simulink library "casper_library_reorder"  (Simulink 7.2)
settings: Solver=ode45  SolverMode=SingleTasking  StartTime=0.0  StopTime=10.0  RelTol=1e-3
libraries: xbsIndex_r4 x122, casper_library_delays x4, xps_library x2, casper_library_bus x2, casper_library_misc x1
(part 1 of 2)
settings Model: Creator=mdexter  LastModifiedBy=davidm

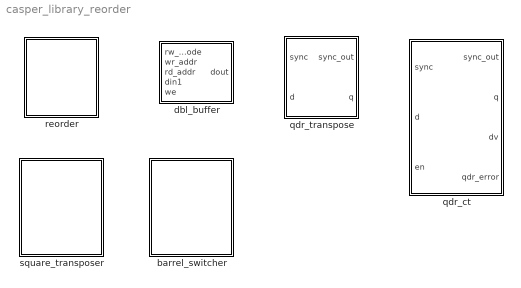
== system casper_library_reorder ==
  barrel_switcher : Subsystem  mask(barrel_switcher){n_inputs=0, async=off}
      mask prompts: n_inputs "Number of Inputs: (2^?)"; async "Asynchronous operation"
      mask help:
      | Shifts input to right by amount specified on sel,
      | wrapping around into higher order bits.
      mask init:
      | barrel_switcher_init(gcb,...
      |     'n_inputs', n_inputs, ...
      |     'async', async);
      mask Help: eval('xlWeb(''http://casper.berkeley.edu/wiki/Barrel_switcher'')')
  dbl_buffer : Subsystem  mask(dbl_buffer){depth=32, latency=2}
  qdr_ct : Subsystem  mask{idepth=10, odepth=7, which_qdr=qdr0, swap_input=no, output_order=in order, step_bits=0, custom_map=[1  15   5   7  10  14   6   0   8   9   2  13  12  11   4   3]}
      mask prompts: idepth "Input vector length (2^?)"; odepth "Output vector length (2^?)"; which_qdr "QDR SRAM chip"; swap_input "Swap input halves?"; output_order "Output column order"; step_bits "Interleave step (2^?)"; custom_map "Custom map"
      mask help:
      | Writes vectors in as rows in matrix and reads
      | out columns. Order in which columns read out
      | determined by 'Output column order' parameter.
      mask init:
      | if (strcmp(output_order, 'interleaved') == 1) && (step_bits > (idepth-1)) ,
      |     errmsg = sprintf('Can''t make step size (%i) bigger than (input vector bit size (%i) - 1)', step_bits, idepth);
      |     errordlg(errmsg);
      | end    
      | 
      | if strcmp(output_order, 'custom') && (...
      |         length(unique(custom_map)) ~= 2^idepth ||...
      |         ~isempty(find(custom_map < 0)) || ...
      |         ~isempty(find(custom_map > (2^idepth)-1))),
      |     disp('Custom map elements must be unique in range 0->2^(input vector)-1');
      |     return;
      | end
      | 
      | % set up output order (in order, interleaved, or custom)
      | map = 0 : (2^idepth)-1;
      | if strcmp(swap_input, 'yes'),
      |     map = [map((length(map)/2)+1:end), map(1:length(map)/2)];
      | end
      | if strcmp(output_order, 'interleaved'),
      |     index = zeros(1, 2^idepth);
      |     step_size = 2^(idepth-step_bits);
      |     for ctr = 0:(2^step_bits)-1,
      |         start = (ctr * step_size) + 1;
      |         finish = start + step_size - 1;
      |         index(start:finish) = ctr+1 : 2^step_bits : 2^idepth;
      |     end
      |     map = map(index);
      |     clear index;
      | elseif strcmp(output_order, 'custom'),
      |     map = map(custom_map+1);
      | end
      | 
      | %generate map so that two samples from same position in 
      | %subsequent input vectors are written into same address
      | map = reshape([map; 2^idepth+map], 1, 2^(idepth+1));
      | 
      | set_param([gcb, '/reorder'], ...
      |     'map', ['[',num2str(map),']']);
      | set_param([gcb, '/qdr'], 'which_qdr', which_qdr);
      mask StyleString: edit,edit,popup(qdr0|qdr1|qdr2|qdr3),popup(no|yes),popup(in order|interleaved|custom),edit,edit
  qdr_transpose : Subsystem  mask{idepth=9, odepth=9, which_qdr=qdr1}
      mask prompts: idepth "Input blocksize (2^n)"; odepth "Output blocksize (2^n)"; which_qdr "QDR Chip"
      mask init:
      | set_param([gcb, '/qdr'], 'which_qdr', which_qdr);
      mask StyleString: edit,edit,popup(qdr0|qdr1|qdr2|qdr3)
  reorder : Subsystem  mask(reorder){map=[], n_bits=0, n_inputs=1, bram_latency=1, map_latency=1, fanout_latency=0, double_buffer=0, bram_map=off}
      mask prompts: map "Output Order:"; n_bits "Data width in"; n_inputs "Number of inputs"; bram_latency "BRAM Latency"; map_latency "Map Latency"; fanout_latency "Fanout latency"; double_buffer "Double Buffer"; bram_map "Use BlockRAM for Map"
      mask init:
      | reorder_init(gcb, ...
      |     'map', map, ...
      |     'n_bits', n_bits, ...
      |     'n_inputs', n_inputs, ...
      |     'bram_latency', bram_latency, ...
      |     'map_latency', map_latency, ...
      |     'fanout_latency', fanout_latency, ...
      |     'double_buffer', double_buffer, ...
      |     'bram_map', bram_map);
      mask Help: eval('xlWeb(''http://casper.berkeley.edu/wiki/Reorder'')')
  square_transposer : Subsystem  mask(square_transposer){n_inputs=0, async=off}
      mask prompts: n_inputs "Number of inputs (2^?):"; async "Aynchronus operation"
      mask init:
      | square_transposer_init(gcb,...
      |     'n_inputs', n_inputs, ...
      |     'async', async);
      mask Help: eval('xlWeb(''http://casper.berkeley.edu/wiki/Square_transposer'')')

== system casper_library_reorder/barrel_switcher ==

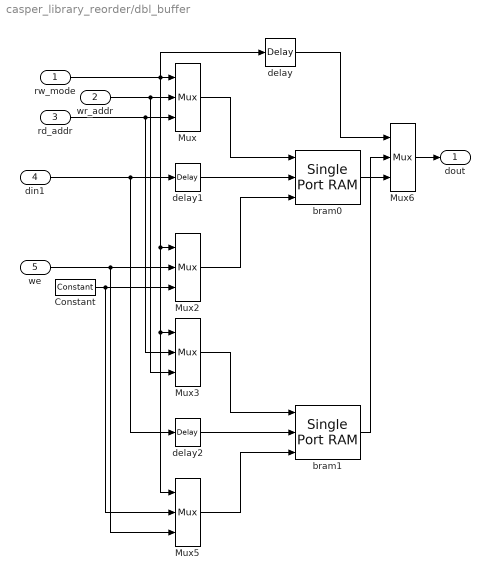
== system casper_library_reorder/dbl_buffer ==
  rw_mode : Inport
  wr_addr : Inport  Port=2
  rd_addr : Inport  Port=3
  din1 : Inport  Port=4
  we : Inport  Port=5
  Constant : xbsIndex_r4/Constant  const=0  gui_display_data_type=Fixed-point  arith_type=Boolean  n_bits=1  bin_pt=0  preci_type=Single  exp_width=8  frac_width=24  explicit_period=on  period=1  equ=P=C  opselect=C  inp2=PCIN>>17  opr=+  inp1=P  carry=CIN  dbl_ovrd=off  block_type=constant
      settings: block_version=9.1.01
  Mux{,2..3,5..6} (5 alike) : xbsIndex_r4/Mux  inputs=2  en=off  latency=1  precision=Full  arith_type="Signed  (2's comp)"  n_bits=8  bin_pt=2  quantization=Truncate  overflow=Wrap  dbl_ovrd=off  block_type=mux
      settings: xl_area=[0, 0, 0, 0, 0, 0, 0]  block_version=9.1.01
  bram0 : xbsIndex_r4/Single Port RAM  depth=depth  initVector=0  distributed_mem=Block RAM  write_mode=Read Before Write  rst=off  init_reg=0  en=off  latency=latency  dbl_ovrd=off  optimize=Area  block_type=spram
      settings: xl_area=[0, 0, 0, 0, 0, 0, 0]  block_version=9.1.01
  bram1 : xbsIndex_r4/Single Port RAM  depth=depth  initVector=0  distributed_mem=Block RAM  write_mode=Read Before Write  rst=off  init_reg=0  en=off  latency=latency  dbl_ovrd=off  optimize=Area  block_type=spram
      settings: xl_area=[0, 0, 0, 0, 0, 0, 0]  block_version=9.1.01
  delay : xbsIndex_r4/Delay  rst=off  infoeditControl=Selection of Reset will increase slice count due to use of real FFs and instead of SRLs  en=off  latency=latency + 1  dbl_ovrd=off  reg_retiming=on  block_type=delay
      settings: xl_area=[0, 0, 0, 0, 0, 0, 0]  block_version=9.1.01
  delay1 : xbsIndex_r4/Delay  rst=off  infoeditControl=Selection of Reset will increase slice count due to use of real FFs and instead of SRLs  en=off  latency=1  dbl_ovrd=off  reg_retiming=on  block_type=delay
      settings: xl_area=[0, 0, 0, 0, 0, 0, 0]  block_version=9.1.01
  delay2 : xbsIndex_r4/Delay  rst=off  infoeditControl=Selection of Reset will increase slice count due to use of real FFs and instead of SRLs  en=off  latency=1  dbl_ovrd=off  reg_retiming=on  block_type=delay
      settings: xl_area=[0, 0, 0, 0, 0, 0, 0]  block_version=9.1.01
  dout : Outport
  wires:
  Constant/1 -> Mux5/2, Mux2/3
  we/1 -> Mux5/3, Mux2/2
  Mux2/1 -> bram0/3
  Mux5/1 -> bram1/3
  Mux6/1 -> dout/1
  delay/1 -> Mux6/1
  din1/1 -> delay2/1, delay1/1
  bram0/1 -> Mux6/3
  bram1/1 -> Mux6/2
  rd_addr/1 -> Mux3/2, Mux/3
  wr_addr/1 -> Mux3/3, Mux/2
  rw_mode/1 -> Mux2/1, Mux5/1, Mux3/1, delay/1, Mux/1
  delay2/1 -> bram1/2
  Mux3/1 -> bram1/1
  delay1/1 -> bram0/2
  Mux/1 -> bram0/1

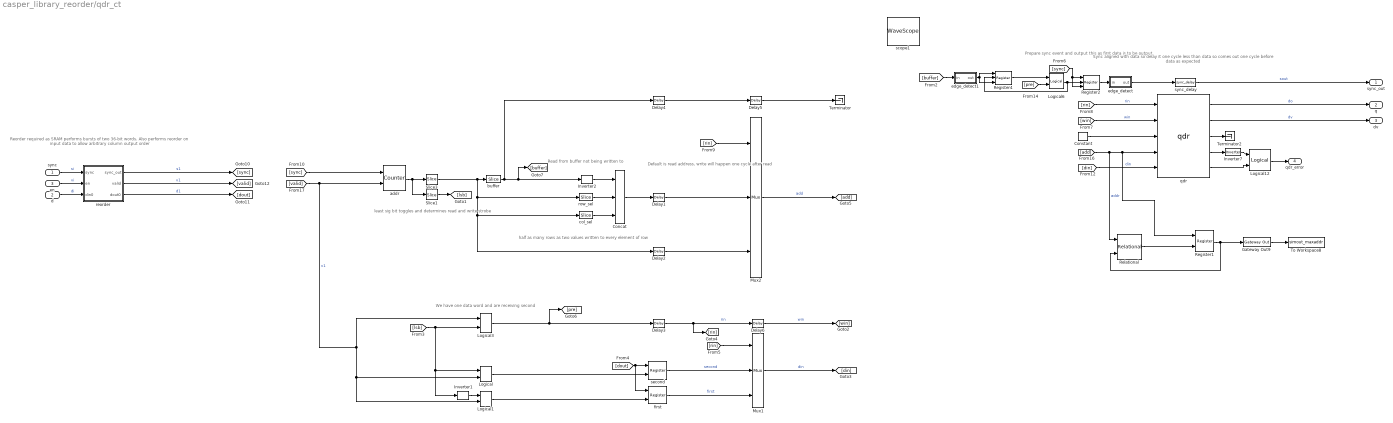
== system casper_library_reorder/qdr_ct ==
  note: Reorder required as SRAM performs
      | bursts of two 36-bit words.
      | Also performs reorder on input
      | data to allow arbitrary column
      | output order
  note: Prepare sync event and output
      | this as first data is to be output.
  note: Sync aligned with data so
      | delay it one cycle less
      | than data so comes out one
      | cycle before data as
      | expected
  note: least sig bit toggles
      | and determines read
      | and write strobe
  note: We have one data word
      | and are receiving second
  note: Default is read address,
      | write will happen one
      | cycle after read
  note: Read from buffer
      | not being
      | written to
  note: half as many rows
      | as two values
      | written to every
      | element of row
  sync : Inport
  d : Inport  Port=2
  en : Inport  Port=3
  Concat : xbsIndex_r4/Concat  num_inputs=3  dbl_ovrd=off  block_type=concat
      settings: block_version=10.1.3
  Constant : xbsIndex_r4/Constant  const=15  gui_display_data_type=Fixed-point  arith_type=Unsigned  n_bits=4  bin_pt=0  preci_type=Single  exp_width=8  frac_width=24  explicit_period=on  period=1  equ=P=C  opselect=C  inp2=PCIN>>17  opr=+  inp1=P  carry=CIN  dbl_ovrd=off  block_type=constant
  Delay{1..6} (6 alike) : xbsIndex_r4/Delay  rst=off  infoeditControl=Selection of Reset will increase slice count due to use of real FFs and instead of SRLs  en=off  latency=1  dbl_ovrd=off  reg_retiming=on  block_type=delay
      settings: block_version=11.4
  Gateway Out9 : xbsIndex_r4/Gateway Out  inherit_from_input=off  hdl_port=off  timing_constraint=None  locs_specified=off  LOCs={}  UseAsDAC=off  DACChannel='1'  block_type=gatewayout
      settings: infoedit="Gateway out block.  Converts Xilinx fixed point inputs into ouputs of type Simulink integer, double, or fixed point.<br><br>Hardware notes:  In hardware these blocks become top level output ports or are discarded, depending on how they are configured."  block_version=11.4
  Inverter1 : xbsIndex_r4/Inverter  en=off  latency=0  dbl_ovrd=off  block_type=inv
  Inverter2 : xbsIndex_r4/Inverter  en=off  latency=0  dbl_ovrd=off  block_type=inv
  Inverter7 : xbsIndex_r4/Inverter  en=off  latency=0  dbl_ovrd=off  block_type=inv
      settings: block_version=11.4
  Logical{,1,3,6} (4 alike) : xbsIndex_r4/Logical  logical_function=AND  inputs=2  en=off  latency=0  precision=Full  arith_type=Unsigned  n_bits=16  bin_pt=0  align_bp=on  dbl_ovrd=off  block_type=logical
      settings: block_version=11.4
  Logical12 : xbsIndex_r4/Logical  logical_function=OR  inputs=2  en=off  latency=1  precision=Full  arith_type=Unsigned  n_bits=8  bin_pt=2  align_bp=on  dbl_ovrd=off  block_type=logical
      settings: xl_area=[0, 0, 0, 0, 0, 0, 0]
  Mux1 : xbsIndex_r4/Mux  inputs=2  en=off  latency=1  precision=Full  arith_type=Unsigned  n_bits=16  bin_pt=14  quantization=Truncate  overflow=Wrap  dbl_ovrd=off  block_type=mux
      settings: block_version=11.4
  Mux2 : xbsIndex_r4/Mux  inputs=2  en=off  latency=1  precision=Full  arith_type=Unsigned  n_bits=16  bin_pt=14  quantization=Truncate  overflow=Wrap  dbl_ovrd=off  block_type=mux
      settings: block_version=11.4
  Register1 : xbsIndex_r4/Register  init=0  rst=off  en=on  dbl_ovrd=off  block_type=register
      settings: block_version=11.4
  Register2 : xbsIndex_r4/Register  init=0  rst=on  en=on  dbl_ovrd=off  block_type=register
      settings: block_version=11.4
  Register4 : xbsIndex_r4/Register  init=0  rst=on  en=on  dbl_ovrd=off  block_type=register
      settings: block_version=11.4
  Relational : xbsIndex_r4/Relational  mode=a>b  en=off  latency=0  dbl_ovrd=off  block_type=relational
  Slice1 : xbsIndex_r4/Slice  nbits=1  boolean_output=on  mode=Lower Bit Location + Width  bit1=0  base1=MSB of Input  bit0=0  base0=LSB of Input  dbl_ovrd=off  block_type=slice
      settings: block_version=10.1.3
  Slice3 : xbsIndex_r4/Slice  nbits=(idepth + odepth + 1) - 1  boolean_output=off  mode=Upper Bit Location + Width  bit1=0  base1=MSB of Input  bit0=0  base0=LSB of Input  dbl_ovrd=off  block_type=slice
      settings: block_version=10.1.3
  Terminator : Terminator
  Terminator2 : Terminator
  To Workspace8 : ToWorkspace  VariableName=simout_maxaddr  SampleTime=-1  SaveFormat=Structure
      settings: MaxDataPoints=1
  addr : xbsIndex_r4/Counter  cnt_type=Free Running  cnt_to=Inf  operation=Up  start_count=0  cnt_by_val=1  arith_type=Unsigned  n_bits=(idepth + odepth + 1)  bin_pt=0  load_pin=off  rst=on  en=on  explicit_period=on  period=1  dbl_ovrd=off  use_behavioral_HDL=on  implementation=Fabric  use_rpm=off  block_type=counter
  buffer : xbsIndex_r4/Slice  nbits=1  boolean_output=on  mode=Upper Bit Location + Width  bit1=0  base1=MSB of Input  bit0=0  base0=LSB of Input  dbl_ovrd=off  block_type=slice
      settings: block_version=10.1.3
  col_sel : xbsIndex_r4/Slice  nbits=idepth  boolean_output=off  mode=Lower Bit Location + Width  bit1=0  base1=MSB of Input  bit0=odepth-1  base0=LSB of Input  dbl_ovrd=off  block_type=slice
      settings: block_version=10.1.3
  edge_detect : Subsystem  AncestorBlock=casper_library_misc/edge_detect  mask(edge_detect){edge=Falling, polarity=Active High, x_in=[0 0.08 0.08 0.16 0.16 0.24 0.24 0.32 0.32 0.4], y_in=[1  1 -1 -1 -1 -1 -1 -1 -1 -1], x_out=[0.6 0.68 0.68 0.76 0.76 0.84 0.84 0.92 0.92 1], y_out=[-1 -1  1  1 -1 -1 -1 -1 -1 -1]}
      mask prompts: edge "Edge Type"; polarity "Output Polarity"; x_in "Input X Positions"; y_in "Input Y Positions"; x_out "Output X Positions"; y_out "Output Y Positions"
      mask help: Output is active for one-cycle after each edge of the specified type (i.e. rising, falling or both).
      mask init:
      | edge_detect_init(gcb,...
      |     'edge',edge,...
      |     'polarity',polarity,...
      |     'x_in',x_in,...
      |     'x_out',x_out,...
      |     'y_in',y_in,...
      |     'y_out',y_out);
      | 
      | x_in_num=str2num(getfield(getfield(get_param(gcb,'UserData'),'parameters'),'x_in'));
      | x_out_num=str2num(getfield(getfield(get_param(gcb,'UserData'),'parameters'),'x_out'));
      | y_in_num=str2num(getfield(getfield(get_param(gcb,'UserData'),'parameters'),'y_in'));
      | y_out_num=str2num(getfield(getfield(get_param(gcb,'UserData'),'parameters'),'y_out'));
      settings: AttributesFormatString=|
      | falling edges
      | active high
      mask Help: Output is active for one-cycle after each edge of the specified type (i.e. rising, falling, or both).  Latency is zero.
      mask StyleString: popup(Rising|Falling|Both),popup(Active High|Active Low),edit,edit,edit,edit
      mask Display:
      | plot(x_in_num,0.5+y_in_num*0.2);
      | plot(x_out_num,0.5+y_out_num*0.2);
  edge_detect1 : Subsystem  AncestorBlock=casper_library_misc/edge_detect  mask(edge_detect){edge=Rising, polarity=Active High, x_in=[0 0.08 0.08 0.16 0.16 0.24 0.24 0.32 0.32 0.4], y_in=[-1 -1  1  1  1  1  1  1  1  1], x_out=[0.6 0.68 0.68 0.76 0.76 0.84 0.84 0.92 0.92 1], y_out=[-1 -1  1  1 -1 -1 -1 -1 -1 -1]}
      mask prompts: edge "Edge Type"; polarity "Output Polarity"; x_in "Input X Positions"; y_in "Input Y Positions"; x_out "Output X Positions"; y_out "Output Y Positions"
      mask help: Output is active for one-cycle after each edge of the specified type (i.e. rising, falling or both).
      mask init: same as casper_library_reorder/qdr_ct/edge_detect
      settings: AttributesFormatString=|
      | rising edges
      | active high
      mask Help: Output is active for one-cycle after each edge of the specified type (i.e. rising, falling, or both).  Latency is zero.
      mask StyleString: popup(Rising|Falling|Both),popup(Active High|Active Low),edit,edit,edit,edit
      mask Display:
      | plot(x_in_num,0.5+y_in_num*0.2);
      | plot(x_out_num,0.5+y_out_num*0.2);
  first : xbsIndex_r4/Register  init=0  rst=off  en=on  dbl_ovrd=off  block_type=register
      settings: block_version=11.4
  qdr : xps_library/qdr  Tag=xps:qdr  which_qdr=qdr0  qdr_awidth=20  use_sniffer=off
  reorder : Subsystem  AncestorBlock=casper_library_reorder/reorder  mask(reorder){map=[0  1024     1  1025     2  1026     3  1027     4  1028     5  1029     6  1030     7  1031     8  1032     9  1033    10  1034    11  1035    12  1036    13  1037    14  1038    15  1039    16  1040    17  1041    18  1042    19  1043    20  1044    21  1045    22  1046    23  1047    24  1048    25  1049    26  1050    27  1051    28  1052    29  1053    30  1054    31  1055    32  1056    33  1057    34  1058    35  1059    36  1060    37  1061    38  1062    39  1063    40  1064    41  1065    42  1066    43  1067    44  1068    45  1069    46  1070    47  1071    48  1072    49  1073    50  1074    51  1075    52  1076    53  1077    54  1078    55  1079    56  1080    57  1081    58  1082    59  1083    60  1084    61  1085    62  1086    63  1087    64  1088    65  1089    66  1090    67  1091    68  1092    69  1093    70  1094    71  1095    72  1096    73  1097    74  1098    75  1099    76  1100    77  1101    78  1102    79  1103    80  1104    81  1105    82  1106    83  1107    84  1108    85  1109    86  1110    87  1111    88  1112    89  1113    90  1114    91  1115    92  1116    93  1117    94  1118    95  1119    96  1120    97  1121    98  1122    99  1123   100  1124   101  1125   102  1126   103  1127   104  1128   105  1129   106  1130   107  1131   108  1132   109  1133   110  1134   111  1135   112  1136   113  1137   114  1138   115  1139   116  1140   117  1141   118  1142   119  1143   120  1144   121  1145   122  1146   123  1147   124  1148   125  1149   126  1150   127  1151   128  1152   129  1153   130  1154   131  1155   132  1156   133  1157   134  1158   135  1159   136  1160   137  1161   138  1162   139  1163   140  1164   141  1165   142  1166   143  1167   144  1168   145  1169   146  1170   147  1171   148  1172   149  1173   150  1174   151  1175   152  1176   153  1177   154  1178   155  1179   156  1180   157  1181   158  1182   159  1183   160  1184   161  1185   162  1186   163  1187   164  1188   165  1189   166  1190   167  1191   168  1192   169  1193   170  1194   171  1195   172  1196   173  1197   174  1198   175  1199   176  1200   177  1201   178  1202   179  1203   180  1204   181  1205   182  1206   183  1207   184  1208   185  1209   186  1210   187  1211   188  1212   189  1213   190  1214   191  1215   192  1216   193  1217   194  1218   195  1219   196  1220   197  1221   198  1222   199  1223   200  1224   201  1225   202  1226   203  1227   204  1228   205  1229   206  1230   207  1231   208  1232   209  1233   210  1234   211  1235   212  1236   213  1237   214  1238   215  1239   216  1240   217  1241   218  1242   219  1243   220  1244   221  1245   222  1246   223  1247   224  1248   225  1249   226  1250   227  1251   228  1252   229  1253   230  1254   231  1255   232  1256   233  1257   234  1258   235  1259   236  1260   237  1261   238  1262   239  1263   240  1264   241  1265   242  1266   243  1267   244  1268   245  1269   246  1270   247  1271   248  1272   249  1273   250  1274   251  1275   252  1276   253  1277   254  1278   255  1279   256  1280   257  1281   258  1282   259  1283   260  1284   261  1285   262  1286   263  1287   264  1288   265  1289   266  1290   267  1291   268  1292   269  1293   270  1294   271  1295   272  1296   273  1297   274  1298   275  1299   276  1300   277  1301   278  1302   279  1303   280  1304   281  1305   282  1306   283  1307   284  1308   285  1309   286  1310   287  1311   288  1312   289  1313   290  1314   291  1315   292  1316   293  1317   294  1318   295  1319   296  1320   297  1321   298  1322   299  1323   300  1324   301  1325   302  1326   303  1327   304  1328   305  1329   306  1330   307  1331   308  1332   309  1333   310  1334   311  1335   312  1336   313  1337   314  1338   315  1339   316  1340   317  1341   318  1342   319  1343   320  1344   321  1345   322  1346   323  1347   324  1348   325  1349   326  1350   327  1351   328  1352   329  1353   330  1354   331  1355   332  1356   333 ...(+8285 chars)], n_bits=0, n_inputs=1, bram_latency=3, map_latency=2, fanout_latency=0, double_buffer=0, bram_map=on}
      mask prompts: map "Output Order:"; n_bits "Data width in"; n_inputs "Number of inputs"; bram_latency "BRAM Latency"; map_latency "Map Latency"; fanout_latency "Fanout latency"; double_buffer "Double Buffer"; bram_map "Use BlockRAM for Map"
      mask init: same as casper_library_reorder/reorder
      settings: AttributesFormatString=order=11
      mask Help: eval('xlWeb(''http://casper.berkeley.edu/wiki/Reorder'')')
  row_sel : xbsIndex_r4/Slice  nbits=odepth-1  boolean_output=off  mode=Lower Bit Location + Width  bit1=0  base1=MSB of Input  bit0=0  base0=LSB of Input  dbl_ovrd=off  block_type=slice
      settings: block_version=10.1.3
  scope1 : xbsIndex_r4/WaveScope  block_type=wavescope
      settings: block_version=11.4
  second : xbsIndex_r4/Register  init=0  rst=off  en=on  dbl_ovrd=off  block_type=register
      settings: block_version=11.4
  sync_delay : casper_library_delays/sync_delay  DelayLen=10-1
  sync_out : Outport
  q : Outport  Port=2
  dv : Outport  Port=3
  qdr_error : Outport  Port=4
  wires:
  sync/1 -> reorder/1(sync)  "si"
  en/1 -> reorder/2(en)  "vi"
  [rin] -> qdr/1  "rin"
  [win] -> qdr/2  "win"
  Constant/1 -> qdr/3
  [add] -> Relational/1, Register1/1, qdr/4  "addr"
  qdr/5 -> Logical12/2
  qdr/4 -> Inverter7/1
  qdr/3 -> Terminator2/1
  addr/1 -> Slice1/1, Slice3/1
  Logical/1 -> second/2
  Logical1/1 -> first/2
  [rin] -> Mux1/1
  Mux1/1 -> [din]  "din"
  [din] -> qdr/5  "din"
  buffer/1 -> [buffer], Inverter2/1, Delay4/1
  [sync] -> Register2/1, Register2/3
  Register4/1 -> Logical6/1
  [pre] -> Logical6/2
  Logical6/1 -> Register2/2, Register4/2
  Register2/1 -> edge_detect/1(in)
  edge_detect/1(out) -> sync_delay/1
  row_sel/1 -> Concat/2
  [rin] -> Mux2/1
  Concat/1 -> Delay1/1
  Inverter2/1 -> Concat/1
  Delay3/1 -> [rin], Delay6/1  "rin"
  [buffer] -> edge_detect1/1(in)
  edge_detect1/1(out) -> Register4/1, Register4/3
  col_sel/1 -> Concat/3
  second/1 -> Mux1/2  "second"
  first/1 -> Mux1/3  "first"
  Delay6/1 -> [win]  "win"
  Logical3/1 -> Delay3/1, [pre]
  Inverter1/1 -> Logical1/1
  Slice3/1 -> buffer/1, row_sel/1, col_sel/1, Delay2/1
  Slice1/1 -> [lsb]
  [lsb] -> Logical3/2, Inverter1/1, Logical/1
  Mux2/1 -> [add]  "add"
  Delay1/1 -> Mux2/2
  Delay2/1 -> Mux2/3
  Delay4/1 -> Delay5/1
  Delay5/1 -> Terminator/1
  [valid] -> addr/2, Logical/2, Logical1/2, Logical3/1  "v1"
  d/1 -> reorder/3(din0)  "di"
  [dout] -> second/1, first/1
  Inverter7/1 -> Logical12/1
  Logical12/1 -> qdr_error/1
  sync_delay/1 -> sync_out/1  "sout"
  qdr/1 -> q/1  "do"
  qdr/2 -> dv/1  "dv"
  Gateway Out9/1 -> To Workspace8/1
  Relational/1 -> Register1/2
  Register1/1 -> Gateway Out9/1, Relational/2
  [sync] -> addr/1
  reorder/1(sync_out) -> [sync]  "s1"
  reorder/2(valid) -> [valid]  "v1"
  reorder/3(dout0) -> [dout]  "d1"

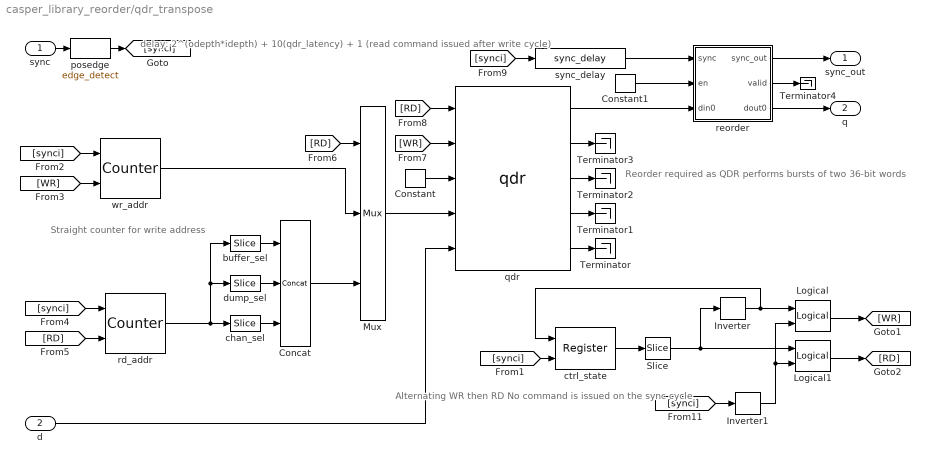
== system casper_library_reorder/qdr_transpose ==
  note: Straight counter for
      | write address
  note: Alternating WR then RD
      | No command is issued
      | on the sync cycle
  note: Reorder required as QDR performs
      | bursts of two 36-bit words
  note: delay: 2^(odepth*idepth) + 10(qdr_latency) + 1
      | (read command issued after write cycle)
  sync : Inport
  d : Inport  Port=2
  Concat : xbsIndex_r4/Concat  num_inputs=3  dbl_ovrd=off  block_type=concat
      settings: block_version=10.1.3
  Constant : xbsIndex_r4/Constant  const=15  gui_display_data_type=Fixed-point  arith_type=Unsigned  n_bits=4  bin_pt=0  preci_type=Single  exp_width=8  frac_width=24  explicit_period=on  period=1  equ=P=C  opselect=C  inp2=PCIN>>17  opr=+  inp1=P  carry=CIN  dbl_ovrd=off  block_type=constant
  Constant1 : xbsIndex_r4/Constant  const=1  gui_display_data_type=Fixed-point  arith_type=Boolean  n_bits=4  bin_pt=0  preci_type=Single  exp_width=8  frac_width=24  explicit_period=on  period=1  equ=P=C  opselect=C  inp2=PCIN>>17  opr=+  inp1=P  carry=CIN  dbl_ovrd=off  block_type=constant
  Inverter : xbsIndex_r4/Inverter  en=off  latency=0  dbl_ovrd=off  block_type=inv
  Inverter1 : xbsIndex_r4/Inverter  en=off  latency=0  dbl_ovrd=off  block_type=inv
  Logical : xbsIndex_r4/Logical  logical_function=AND  inputs=2  en=off  latency=0  precision=Full  arith_type=Unsigned  n_bits=16  bin_pt=0  align_bp=on  dbl_ovrd=off  block_type=logical
  Logical1 : xbsIndex_r4/Logical  logical_function=AND  inputs=2  en=off  latency=0  precision=Full  arith_type=Unsigned  n_bits=16  bin_pt=0  align_bp=on  dbl_ovrd=off  block_type=logical
  Mux : xbsIndex_r4/Mux  inputs=2  en=off  latency=0  precision=Full  arith_type=Unsigned  n_bits=16  bin_pt=14  quantization=Truncate  overflow=Wrap  dbl_ovrd=off  block_type=mux
  Slice : xbsIndex_r4/Slice  nbits=1  boolean_output=on  mode=Lower Bit Location + Width  bit1=0  base1=MSB of Input  bit0=0  base0=LSB of Input  dbl_ovrd=off  block_type=slice
      settings: infoedit="Extracts a given range of bits from each input sample and presents it at the output.  The output type is ordinarily unsigned with binary point at zero, but can be Boolean when the slice is one bit wide.<P><P>Hardware notes: In hardware this block costs nothing."  block_version=10.1.3
  Terminator{,1..4} (5 alike) : Terminator
  buffer_sel : xbsIndex_r4/Slice  nbits=1  boolean_output=off  mode=Upper Bit Location + Width  bit1=0  base1=MSB of Input  bit0=0  base0=LSB of Input  dbl_ovrd=off  block_type=slice
      settings: infoedit="Extracts a given range of bits from each input sample and presents it at the output.  The output type is ordinarily unsigned with binary point at zero, but can be Boolean when the slice is one bit wide.<P><P>Hardware notes: In hardware this block costs nothing."  block_version=10.1.3
  chan_sel : xbsIndex_r4/Slice  nbits=idepth - 1  boolean_output=off  mode=Lower Bit Location + Width  bit1=9-1  base1=MSB of Input  bit0=odepth  base0=LSB of Input  dbl_ovrd=off  block_type=slice
      settings: infoedit="Extracts a given range of bits from each input sample and presents it at the output.  The output type is ordinarily unsigned with binary point at zero, but can be Boolean when the slice is one bit wide.<P><P>Hardware notes: In hardware this block costs nothing."  block_version=10.1.3
  ctrl_state : xbsIndex_r4/Register  init=0  rst=on  en=off  dbl_ovrd=off  block_type=register
  dump_sel : xbsIndex_r4/Slice  nbits=odepth  boolean_output=off  mode=Lower Bit Location + Width  bit1=0  base1=MSB of Input  bit0=0  base0=LSB of Input  dbl_ovrd=off  block_type=slice
      settings: infoedit="Extracts a given range of bits from each input sample and presents it at the output.  The output type is ordinarily unsigned with binary point at zero, but can be Boolean when the slice is one bit wide.<P><P>Hardware notes: In hardware this block costs nothing."  block_version=10.1.3
  posedge : casper_library_misc/edge_detect  edge=Rising  polarity=Active High  x_in=[0 0.08 0.08 0.16 0.16 0.24 0.24 0.32 0.32 0.4]  y_in="[-1 -1  1  1  1  1  1  1  1  1]"  x_out=[0.6 0.68 0.68 0.76 0.76 0.84 0.84 0.92 0.92 1]  y_out="[-1 -1  1  1 -1 -1 -1 -1 -1 -1]"
  qdr : xps_library/qdr  Tag=xps:qdr  which_qdr=qdr1  qdr_awidth=odepth+idepth+1  use_sniffer=off
  rd_addr : xbsIndex_r4/Counter  cnt_type=Free Running  cnt_to=Inf  operation=Up  start_count=2^(odepth + idepth - 1)  cnt_by_val=1  arith_type=Unsigned  n_bits=(idepth + odepth + 1) - 1  bin_pt=0  load_pin=off  rst=on  en=on  explicit_period=on  period=1  dbl_ovrd=off  use_behavioral_HDL=on  implementation=Fabric  use_rpm=off  block_type=counter
  reorder : Subsystem  AncestorBlock=casper_library_reorder/reorder  mask(reorder){map=[[0:2^odepth-1]*2 [0:2^odepth-1]*2 + 1], n_bits=0, n_inputs=1, bram_latency=2, map_latency=3, fanout_latency=0, double_buffer=0, bram_map=off}
      mask prompts: map "Output Order:"; n_bits "Data width in"; n_inputs "Number of inputs"; bram_latency "BRAM Latency"; map_latency "Map Latency"; fanout_latency "Fanout latency"; double_buffer "Double Buffer"; bram_map "Use BlockRAM for Map"
      mask init: same as casper_library_reorder/reorder
      settings: AttributesFormatString=order=10
      mask Help: eval('xlWeb(''http://casper.berkeley.edu/wiki/Reorder'')')
  sync_delay : casper_library_delays/sync_delay  DelayLen=2^(idepth + odepth) + 10 + 1
  wr_addr : xbsIndex_r4/Counter  cnt_type=Free Running  cnt_to=Inf  operation=Up  start_count=0  cnt_by_val=1  arith_type=Unsigned  n_bits=(idepth + odepth + 1) - 1  bin_pt=0  load_pin=off  rst=on  en=on  explicit_period=on  period=1  dbl_ovrd=off  use_behavioral_HDL=on  implementation=Fabric  use_rpm=off  block_type=counter
  sync_out : Outport
  q : Outport  Port=2
  wires:
  reorder/3(dout0) -> q/1
  reorder/2(valid) -> Terminator4/1
  reorder/1(sync_out) -> sync_out/1
  qdr/1 -> reorder/3(din0)
  Constant1/1 -> reorder/2(en)
  sync_delay/1 -> reorder/1(sync)
  chan_sel/1 -> Concat/3
  dump_sel/1 -> Concat/2
  rd_addr/1 -> dump_sel/1, buffer_sel/1, chan_sel/1
  buffer_sel/1 -> Concat/1
  Concat/1 -> Mux/3
  Logical/1 -> [WR]
  Inverter1/1 -> Logical1/2, Logical/2
  Logical1/1 -> [RD]
  posedge/1 -> [synci]
  [synci] -> Inverter1/1
  Slice/1 -> Logical1/1, Inverter/1
  [synci] -> sync_delay/1
  qdr/2 -> Terminator3/1
  qdr/3 -> Terminator2/1
  qdr/4 -> Terminator1/1
  qdr/5 -> Terminator/1
  d/1 -> qdr/5
  Mux/1 -> qdr/4
  Constant/1 -> qdr/3
  [WR] -> qdr/2
  [RD] -> qdr/1
  wr_addr/1 -> Mux/2
  [RD] -> Mux/1
  Inverter/1 -> Logical/1, ctrl_state/1
  [RD] -> rd_addr/2
  [synci] -> rd_addr/1
  [WR] -> wr_addr/2
  [synci] -> wr_addr/1
  [synci] -> ctrl_state/2
  sync/1 -> posedge/1
  ctrl_state/1 -> Slice/1

== system casper_library_reorder/reorder ==

== system casper_library_reorder/square_transposer ==

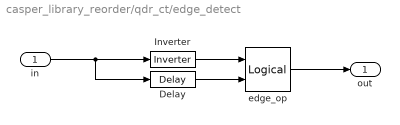
== system casper_library_reorder/qdr_ct/edge_detect ==
  in : Inport
  Delay : xbsIndex_r4/Delay  rst=off  infoeditControl=Selection of Reset will increase slice count due to use of real FFs and instead of SRLs  en=off  latency=1  dbl_ovrd=off  reg_retiming=on  block_type=delay
      settings: xl_area=[0, 0, 0, 0, 0, 0, 0]
  Inverter : xbsIndex_r4/Inverter  en=off  latency=0  dbl_ovrd=off  block_type=inv
      settings: xl_area=[0, 0, 0, 0, 0, 0, 0]
  edge_op : xbsIndex_r4/Logical  logical_function=AND  inputs=2  en=off  latency=0  precision=Full  arith_type=Unsigned  n_bits=8  bin_pt=2  align_bp=on  dbl_ovrd=off  block_type=logical
      settings: xl_area=[0, 0, 0, 0, 0, 0, 0]
  out : Outport
  wires:
  Inverter/1 -> edge_op/1
  edge_op/1 -> out/1
  in/1 -> Inverter/1, Delay/1
  Delay/1 -> edge_op/2

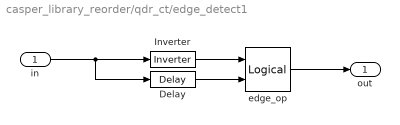
== system casper_library_reorder/qdr_ct/edge_detect1 ==
  in : Inport
  Delay : xbsIndex_r4/Delay  rst=off  infoeditControl=Selection of Reset will increase slice count due to use of real FFs and instead of SRLs  en=off  latency=1  dbl_ovrd=off  reg_retiming=on  block_type=delay
      settings: xl_area=[0, 0, 0, 0, 0, 0, 0]
  Inverter : xbsIndex_r4/Inverter  en=off  latency=0  dbl_ovrd=off  block_type=inv
      settings: xl_area=[0, 0, 0, 0, 0, 0, 0]
  edge_op : xbsIndex_r4/Logical  logical_function=NOR  inputs=2  en=off  latency=0  precision=Full  arith_type=Unsigned  n_bits=8  bin_pt=2  align_bp=on  dbl_ovrd=off  block_type=logical
      settings: xl_area=[0, 0, 0, 0, 0, 0, 0]
  out : Outport
  wires:
  Delay/1 -> edge_op/2
  in/1 -> Delay/1, Inverter/1
  edge_op/1 -> out/1
  Inverter/1 -> edge_op/1
